simulink model "Adaptive_fuzzy_NTSMC"  (R2026a)
settings: Solver=FixedStepAuto  StopTime=150  FixedStep=0.005
values from neighbouring files (symbols this model uses):
  a1 = (Iy-Iz)/Ix    (= -0.733333333333)    [Initialization_3_Torque_Force.m]
  a2 = Jr/Ix    (= 0.008)    [Initialization_3_Torque_Force.m]
  a3 = (Iz-Ix)/Iy    (= 0.733333333333)    [Initialization_3_Torque_Force.m]
  a4 = Jr/Iy    (= 0.008)    [Initialization_3_Torque_Force.m]
  a5 = (Ix-Iy)/Iz    (= 0)    [Initialization_3_Torque_Force.m]
  beta_phi = beta    (= 2.5)    [Initialization_3_Torque_Force.m]
  beta_psi = beta    (= 2.5)    [Initialization_3_Torque_Force.m]
  beta_theta = beta    (= 2.5)    [Initialization_3_Torque_Force.m]
  distFactor = 19.0    (= 19)    [Initialization_3_Torque_Force.m]
  distMode = 3    [Initialization_3_Torque_Force.m]
  g = 9.8    [Initialization_3_Torque_Force.m]
  gama = 1.5    [Initialization_3_Torque_Force.m]
  Ix = 7.5e-3    (= 0.0075)    [Initialization_3_Torque_Force.m]
  Iy = 7.5e-3    (= 0.0075)    [Initialization_3_Torque_Force.m]
  Iz = 1.3e-2    (= 0.013)    [Initialization_3_Torque_Force.m]
  k_psi1 = 10    [Initialization_3_Torque_Force.m]
  k_psi2 = 10    [Initialization_3_Torque_Force.m]
  kd_x = -4    [Initialization_3_Torque_Force.m]
  kd_y = -4    [Initialization_3_Torque_Force.m]
  kd_z = -18    [Initialization_3_Torque_Force.m]
  kp_x = -3    [Initialization_3_Torque_Force.m]
  kp_y = -3    [Initialization_3_Torque_Force.m]
  kp_z = -12    [Initialization_3_Torque_Force.m]
  mass = 0.65    [Initialization_3_Torque_Force.m]
  ro = 0.3    [Initialization_3_Torque_Force.m]
  slctr = 3    [Initialization_3_Torque_Force.m]
  Tfinal = 150    [Initialization_3_Torque_Force.m]
  U2Omega = inv(Omega2U)    [Initialization_3_Torque_Force.m]
  w = [1 1 0.5]    [Initialization_3_Torque_Force.m]
  X0 = [10 10 5]    [Initialization_3_Torque_Force.m]
libraries: simulink x15, fuzblock x2, shared6dof x1
settings Model: Creator=elecomp  LastModifiedBy=asus

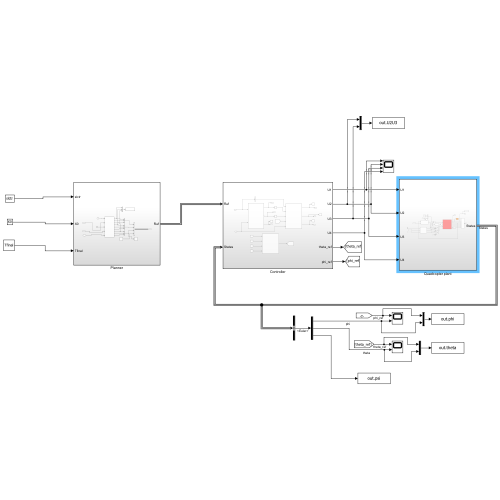
[thumbnail: Simulink's stored preview of the top-level diagram]
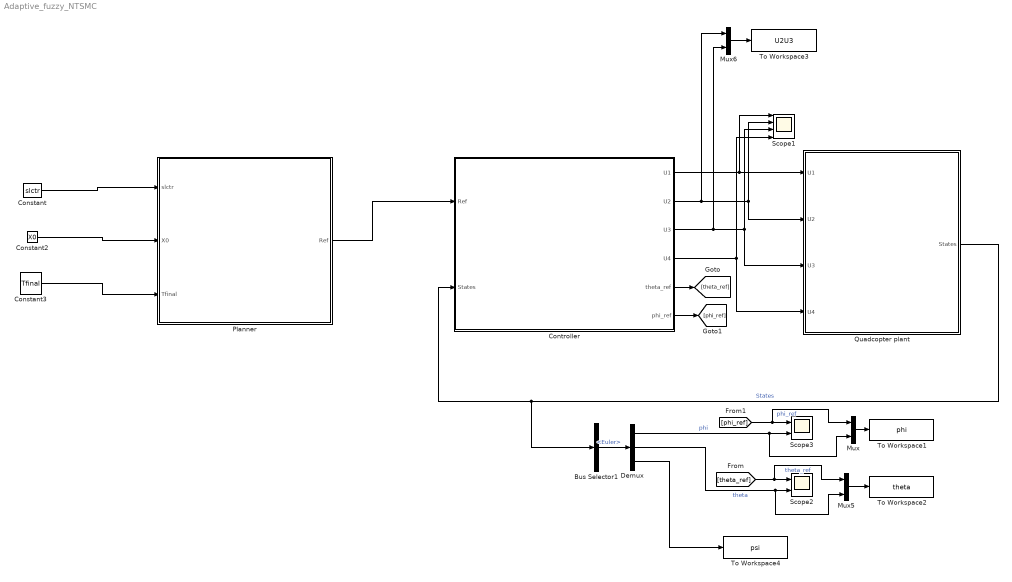
== system Adaptive_fuzzy_NTSMC ==
  Bus Selector1 : BusSelector  OutputSignals=Euler
  Constant : Constant  Value=slctr
  Constant2 : Constant  Value=X0
  Constant3 : Constant  Value=Tfinal
  Controller : Subsystem
  Demux : Demux  Outputs=3
  Mux : Mux  Inputs=2
  Mux5 : Mux  Inputs=2
  Mux6 : Mux  Inputs=2
  Planner : Subsystem
  Quadcopter plant : Subsystem
  Scope1 : Scope  NumInputPorts=4
      settings: ActiveDisplayYMinimum=-2.18019  ActiveDisplayYMaximum=1.22126  DataLoggingVariableName=ScopeData2
  Scope2 : Scope  NumInputPorts=2
      settings: ActiveDisplayYMinimum=-1.95741  ActiveDisplayYMaximum=1.91397
  Scope3 : Scope  NumInputPorts=2
      settings: ActiveDisplayYMinimum=-0.55732  ActiveDisplayYMaximum=1.11824  DataLoggingVariableName=ScopeData2
  To Workspace1 : ToWorkspace  VariableName=phi  SaveFormat=Timeseries  SampleTime=-1
  To Workspace2 : ToWorkspace  VariableName=theta  SaveFormat=Timeseries  SampleTime=-1
  To Workspace3 : ToWorkspace  VariableName=U2U3  SaveFormat=Timeseries  SampleTime=-1
  To Workspace4 : ToWorkspace  VariableName=psi  SaveFormat=Timeseries  SampleTime=-1
  wires:
  Quadcopter plant/1(States) -> Bus Selector1/1, Controller/2(States)  "States"
  Controller/1(U1) -> Scope1/1, Quadcopter plant/1(U1)
  Controller/2(U2) -> Mux6/1, Quadcopter plant/2(U2), Scope1/2
  Controller/3(U3) -> Mux6/2, Quadcopter plant/3(U3), Scope1/3
  Controller/4(U4) -> Quadcopter plant/4(U4), Scope1/4
  Bus Selector1/1 -> Demux/1  "<Euler>"
  Demux/2 -> Mux5/2, Scope2/2  "theta"
  Demux/1 -> Mux/2, Scope3/2  "phi"
  Controller/5(theta_ref) -> [theta_ref]
  Controller/6(phi_ref) -> [phi_ref]
  [theta_ref] -> Mux5/1, Scope2/1  "theta_ref"
  [phi_ref] -> Mux/1, Scope3/1  "phi_ref"
  Mux5/1 -> To Workspace2/1
  Mux/1 -> To Workspace1/1
  Mux6/1 -> To Workspace3/1
  Demux/3 -> To Workspace4/1
  Constant/1 -> Planner/1(slctr)
  Constant2/1 -> Planner/2(X0)
  Constant3/1 -> Planner/3(Tfinal)
  Planner/1(Ref) -> Controller/1(Ref)

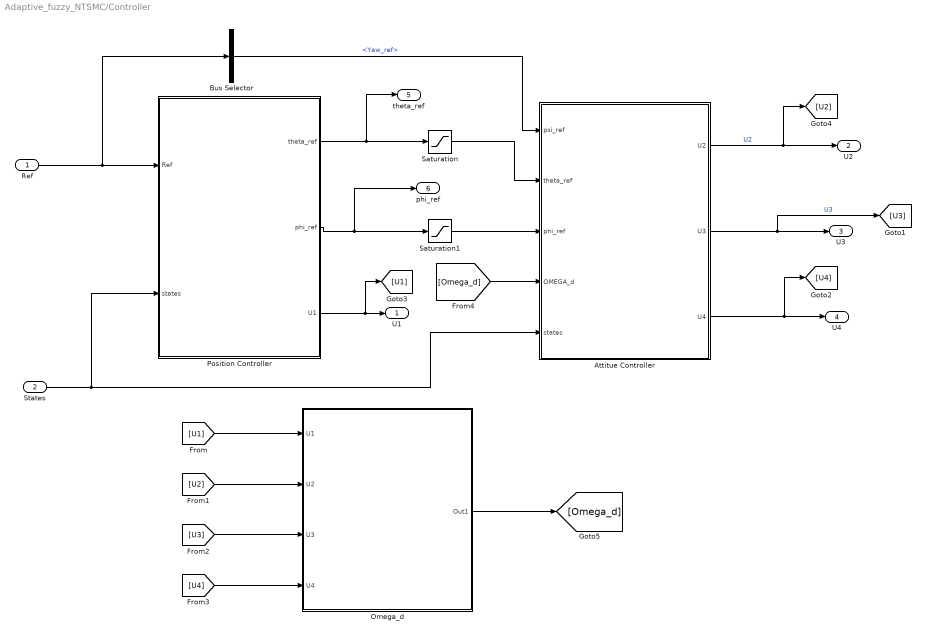
== system Adaptive_fuzzy_NTSMC/Controller ==
  Ref : Inport
  States : Inport  Port=2
  Attitue Controller : Subsystem
  Bus Selector : BusSelector  OutputSignals=Yaw_ref
  Omega_d : Subsystem
  Position Controller : Subsystem
  Saturation : Saturate  UpperLimit=0.7  LowerLimit=-0.7
  Saturation1 : Saturate  UpperLimit=0.7  LowerLimit=-0.7
  U1 : Outport
  U2 : Outport  Port=2
  U3 : Outport  Port=3
  U4 : Outport  Port=4
  theta_ref : Outport  Port=5
  phi_ref : Outport  Port=6
  wires:
  Ref/1 -> Bus Selector/1, Position Controller/1(Ref)
  Position Controller/3(U1) -> [U1], U1/1
  [Omega_d] -> Attitue Controller/4(OMEGA_d)
  Attitue Controller/1(U2) -> [U2], U2/1  "U2"
  Attitue Controller/2(U3) -> [U3], U3/1  "U3"
  Bus Selector/1 -> Attitue Controller/1(psi_ref)  "<Yaw_ref>"
  Attitue Controller/3(U4) -> [U4], U4/1
  Omega_d/1(Out1) -> [Omega_d]
  [U1] -> Omega_d/1(U1)
  [U2] -> Omega_d/2(U2)
  [U3] -> Omega_d/3(U3)
  [U4] -> Omega_d/4(U4)
  Position Controller/1(theta_ref) -> Saturation/1, theta_ref/1
  Position Controller/2(phi_ref) -> Saturation1/1, phi_ref/1
  States/1 -> Attitue Controller/5(states), Position Controller/2(states)
  Saturation/1 -> Attitue Controller/2(theta_ref)
  Saturation1/1 -> Attitue Controller/3(phi_ref)

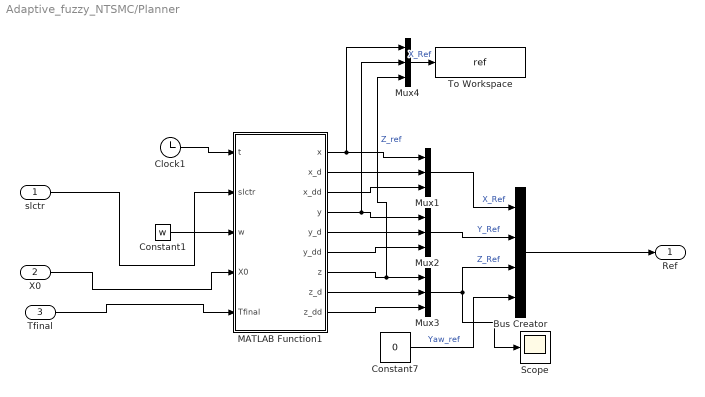
== system Adaptive_fuzzy_NTSMC/Planner ==
  slctr : Inport
  X0 : Inport  Port=2
  Tfinal : Inport  Port=3
  Bus Creator : BusCreator  Inputs=4
  Clock1 : Clock
  Constant1 : Constant  Value=w
  Constant7 : Constant  Value=0
  MATLAB Function1 : MATLAB Function  TreatAsAtomicUnit=on
  Mux{1..4} (4 alike) : Mux  Inputs=3
  Scope : Scope
      settings: ActiveDisplayYMinimum=-0.625  ActiveDisplayYMaximum=5.625
  To Workspace : ToWorkspace  VariableName=ref  SaveFormat=Timeseries  SampleTime=-1
  Ref : Outport
  wires:
  Constant7/1 -> Bus Creator/4  "Yaw_ref"
  MATLAB Function1/1(x) -> Mux4/1, Mux1/1
  MATLAB Function1/6(y_dd) -> Mux2/3
  MATLAB Function1/4(y) -> Mux4/2, Mux2/1
  Mux1/1 -> Bus Creator/1  "X_Ref"
  Mux3/1 -> Bus Creator/3, Scope/1  "Z_Ref"
  MATLAB Function1/3(x_dd) -> Mux1/3
  MATLAB Function1/7(z) -> Mux4/3, Mux3/1  "Z_ref"
  MATLAB Function1/9(z_dd) -> Mux3/3
  Bus Creator/1 -> Ref/1
  slctr/1 -> MATLAB Function1/2(slctr)
  Constant1/1 -> MATLAB Function1/3(w)
  Clock1/1 -> MATLAB Function1/1(t)
  MATLAB Function1/8(z_d) -> Mux3/2
  MATLAB Function1/2(x_d) -> Mux1/2
  Mux4/1 -> To Workspace/1  "X_Ref"
  MATLAB Function1/5(y_d) -> Mux2/2
  Mux2/1 -> Bus Creator/2  "Y_Ref"
  X0/1 -> MATLAB Function1/4(X0)
  Tfinal/1 -> MATLAB Function1/5(Tfinal)

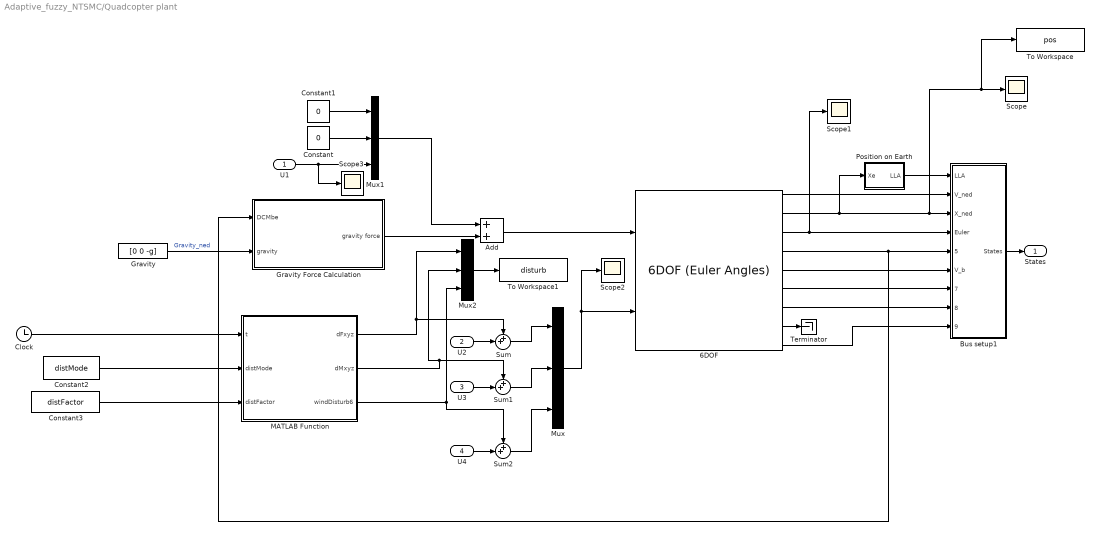
== system Adaptive_fuzzy_NTSMC/Quadcopter plant ==
  U1 : Inport
  U2 : Inport  Port=2
  U3 : Inport  Port=3
  U4 : Inport  Port=4
  "6DOF " : shared6dof/6DOF (Euler Angles)  units=Metric (MKS)  mtype=Fixed  rep=Euler Angles  xme_0=initpos  Vm_0=initvb  eul_0=initeuler  pm_0=initangRates  mass_0=mass  mass_e=0.5  mass_f=2.0  inertia=inertia_mat  inertia_e=eye(3)  inertia_f=2*eye(3)  k_quat=Vehicle.SixDOF.quatGain  vre_flag=on  abi_flag=on  aMode=aMode  xme_statename=''  Vm_statename=''  eul_statename=''  quat_statename=''  pm_statename=''  mass_statename=''
  Add : Sum
  Bus setup1 : Subsystem
  Clock : Clock
  Constant : Constant  Value=0
  Constant1 : Constant  Value=0
  Constant2 : Constant  Value=distMode
  Constant3 : Constant  Value=distFactor
  Gravity : Constant  Value=[0 0 -g]
  Gravity Force Calculation : Subsystem
  MATLAB Function : MATLAB Function  TreatAsAtomicUnit=on
  Mux : Mux  Inputs=3
  Mux1 : Mux  Inputs=3
  Mux2 : Mux  Inputs=3
  Position on Earth : Subsystem  Priority=1  TreatAsAtomicUnit=on
  Scope{,1..3} (4 alike) : Scope
      Scope settings: ActiveDisplayYMinimum=-12.55453  ActiveDisplayYMaximum=12.50157
      Scope1 settings: ActiveDisplayYMinimum=-0.86207  ActiveDisplayYMaximum=0.72361  DataLoggingVariableName=ScopeData4
      Scope2 settings: ActiveDisplayYMinimum=-0.018  ActiveDisplayYMaximum=0.05893  DataLoggingVariableName=ScopeData5
      Scope3 settings: ActiveDisplayYMinimum=-0.08846  ActiveDisplayYMaximum=0.08533
  Sum : Sum  Inputs=++|
  Sum1 : Sum  Inputs=++|
  Sum2 : Sum  Inputs=++|
  Terminator : Terminator
  To Workspace : ToWorkspace  VariableName=pos  SaveFormat=Timeseries  SampleTime=-1
  To Workspace1 : ToWorkspace  VariableName=disturb  SaveFormat=Timeseries  SampleTime=-1
  States : Outport
  wires:
  "6DOF "/4 -> Bus setup1/5(DCM_be), Gravity Force Calculation/1(DCMbe)
  Bus setup1/1(States) -> States/1
  "6DOF "/8 -> Terminator/1
  Gravity/1 -> Gravity Force Calculation/2(gravity)  "Gravity_ned"
  Mux/1 -> Scope2/1, "6DOF "/2
  U1/1 -> Scope3/1, Mux1/3
  Constant/1 -> Mux1/2
  Constant1/1 -> Mux1/1
  Gravity Force Calculation/1(gravity force) -> Add/2
  Mux1/1 -> Add/1
  Add/1 -> "6DOF "/1
  "6DOF "/1 -> Bus setup1/2(V_ned)
  "6DOF "/2 -> Position on Earth/1(Xe), To Workspace/1, Scope/1, Bus setup1/3(X_ned)
  "6DOF "/3 -> Bus setup1/4(Euler), Scope1/1
  "6DOF "/5 -> Bus setup1/6(V_b)
  "6DOF "/6 -> Bus setup1/7(Omega_b)
  "6DOF "/7 -> Bus setup1/8(dOmega_b)
  "6DOF "/9 -> Bus setup1/9(Accel_b)
  Position on Earth/1(LLA) -> Bus setup1/1(LLA)
  U4/1 -> Sum2/2
  U3/1 -> Sum1/2
  U2/1 -> Sum/2
  Sum/1 -> Mux/1
  Sum1/1 -> Mux/2
  Sum2/1 -> Mux/3
  MATLAB Function/3(windDisturb6) -> Sum2/1, Mux2/3
  Mux2/1 -> To Workspace1/1
  MATLAB Function/1(dFxyz) -> Mux2/1, Sum/1
  MATLAB Function/2(dMxyz) -> Mux2/2, Sum1/1
  Clock/1 -> MATLAB Function/1(t)
  Constant3/1 -> MATLAB Function/3(distFactor)
  Constant2/1 -> MATLAB Function/2(distMode)

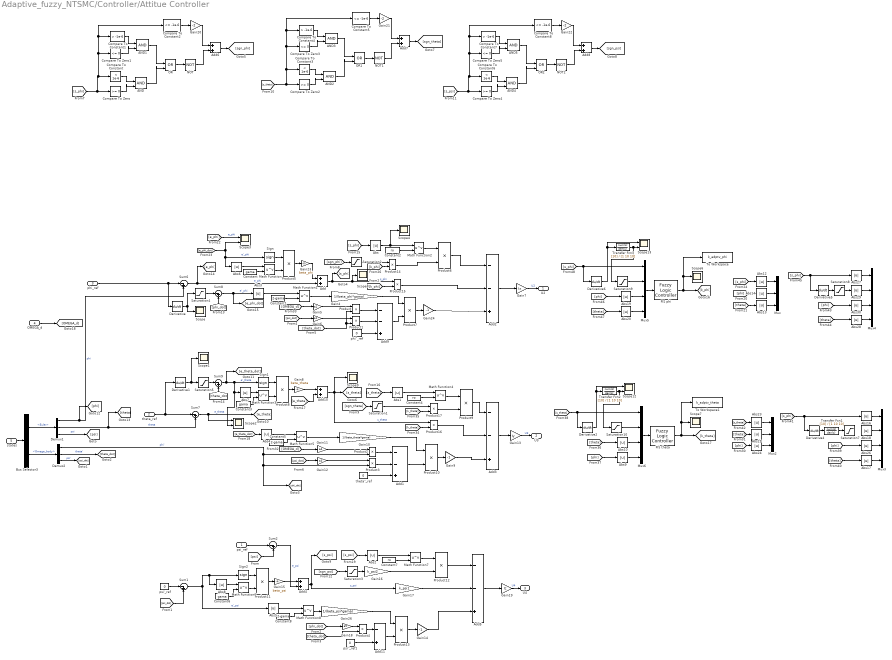
== system Adaptive_fuzzy_NTSMC/Controller/Attitue Controller ==
  psi_ref : Inport
  theta_ref : Inport  Port=2
  phi_ref : Inport  Port=3
  OMEGA_d : Inport  Port=4
  states : Inport  Port=5
  AND{,1..5} (6 alike) : Logic  IconShape=distinctive  AllPortsSameDT=off  OutDataTypeStr=boolean
  Abs{,1..10,12..14,16..20,23..30} (27 alike) : Abs  SaturateOnIntegerOverflow=off
  Add{,4,6..8,10} (6 alike) : Sum
  Add{1..3,5,9} (5 alike) : Sum  Inputs=--+
  Add11 : Sum  Inputs=-+
  Bus Selector3 : BusSelector  OutputSignals=Euler,Omega_body
  Compare To Constant : simulink/Logic and Bit Operations/Compare To Constant  relop=<  const=1e-6  OutDataTypeStr=boolean
  Compare To Constant1 : simulink/Logic and Bit Operations/Compare To Constant  relop=>  const=-1e-6  OutDataTypeStr=boolean
  Compare To Constant2 : simulink/Logic and Bit Operations/Compare To Constant  relop=<=  const=-1e-6  OutDataTypeStr=boolean
  Compare To Constant3 : simulink/Logic and Bit Operations/Compare To Constant  relop=<  const=1e-6  OutDataTypeStr=boolean
  Compare To Constant4 : simulink/Logic and Bit Operations/Compare To Constant  relop=>  const=-1e-6  OutDataTypeStr=boolean
  Compare To Constant5 : simulink/Logic and Bit Operations/Compare To Constant  relop=<=  const=-1e-6  OutDataTypeStr=boolean
  Compare To Constant6 : simulink/Logic and Bit Operations/Compare To Constant  relop=<  const=1e-6  OutDataTypeStr=boolean
  Compare To Constant7 : simulink/Logic and Bit Operations/Compare To Constant  relop=>  const=-1e-6  OutDataTypeStr=boolean
  Compare To Constant8 : simulink/Logic and Bit Operations/Compare To Constant  relop=<=  const=-1e-6  OutDataTypeStr=boolean
  Compare To Zero : simulink/Logic and Bit Operations/Compare To Zero  relop=>=  OutDataTypeStr=boolean
  Compare To Zero1 : simulink/Logic and Bit Operations/Compare To Zero  relop=<=  OutDataTypeStr=boolean
  Compare To Zero2 : simulink/Logic and Bit Operations/Compare To Zero  relop=>=  OutDataTypeStr=boolean
  Compare To Zero3 : simulink/Logic and Bit Operations/Compare To Zero  relop=<=  OutDataTypeStr=boolean
  Compare To Zero4 : simulink/Logic and Bit Operations/Compare To Zero  relop=>=  OutDataTypeStr=boolean
  Compare To Zero5 : simulink/Logic and Bit Operations/Compare To Zero  relop=<=  OutDataTypeStr=boolean
  Constant : Constant  Value=gama
  Constant1 : Constant  Value=2-gama
  Constant2 : Constant  Value=ro
  Constant3 : Constant  Value=gama
  Constant4 : Constant  Value=ro
  Constant5 : Constant  Value=2-gama
  Constant6 : Constant  Value=gama
  Constant7 : Constant  Value=ro
  Constant8 : Constant  Value=2-gama
  Demux1 : Demux  Outputs=3
  Demux2 : Demux  Outputs=3
  Derivative{,1..2,4..6} (6 alike) : Derivative
  FIS phi : fuzblock/Fuzzy Logic  Controller  FIS=fis_phi  OutputSampleNumber=101  DataType=double  UseLookupTable=off  NumBreakpoints=10  FuzzifiedInputs=off  RuleFiringStrengths=off  RuleOutputs=off  AggregatedOutputs=off  SimulateUsing=Interpreted execution  OutOfRangeInputValueMessage=warning  NoRuleFiredMessage=warning  EmptyOutputFuzzySetMessage=warning
  FIS theta : fuzblock/Fuzzy Logic  Controller  FIS=fis_theta  OutputSampleNumber=101  DataType=double  UseLookupTable=off  NumBreakpoints=10  FuzzifiedInputs=off  RuleFiringStrengths=off  RuleOutputs=off  AggregatedOutputs=off  SimulateUsing=Interpreted execution  OutOfRangeInputValueMessage=warning  NoRuleFiredMessage=warning  EmptyOutputFuzzySetMessage=warning
  Gain10 : Gain  Gain=1/(beta_theta*gama)
  Gain11 : Gain  Gain=a4
  Gain12 : Gain  Gain=a3
  Gain13 : Gain  Gain=Iy
  Gain14 : Gain  Gain=-1
  Gain15 : Gain  Gain=beta_psi
  Gain16 : Gain  Gain=k_psi2
  Gain17 : Gain  Gain=k_psi1
  Gain18 : Gain  Gain=a5
  Gain19 : Gain  Gain=Iz
  Gain20 : Gain  Gain=-2
  Gain21 : Gain  Gain=-2
  Gain22 : Gain  Gain=-2
  Gain23 : Gain  Gain=beta_phi
  Gain24 : Gain  Gain=-1
  Gain26 : Gain  Gain=1/(beta_psi*gama)
  Gain4 : Gain  Gain=1/(beta_phi*gama)
  Gain5 : Gain  Gain=a2
  Gain6 : Gain  Gain=a1
  Gain7 : Gain  Gain=Ix
  Gain8 : Gain  Gain=beta_theta
  Gain9 : Gain  Gain=-1
  Math Function{,1..8} (9 alike) : Math  Operator=pow
  Mux : Mux  Inputs=3
  Mux2 : Mux  Inputs=3
  Mux{3..6} (4 alike) : Mux
  NOT : Logic  Operator=NOT  IconShape=distinctive  AllPortsSameDT=off  OutDataTypeStr=boolean
  NOT1 : Logic  Operator=NOT  IconShape=distinctive  AllPortsSameDT=off  OutDataTypeStr=boolean
  NOT2 : Logic  Operator=NOT  IconShape=distinctive  AllPortsSameDT=off  OutDataTypeStr=boolean
  OR : Logic  Operator=OR  IconShape=distinctive  AllPortsSameDT=off  OutDataTypeStr=boolean
  OR1 : Logic  Operator=OR  IconShape=distinctive  AllPortsSameDT=off  OutDataTypeStr=boolean
  OR2 : Logic  Operator=OR  IconShape=distinctive  AllPortsSameDT=off  OutDataTypeStr=boolean
  Product{,1..17} (18 alike) : Product
  Saturation1 : Saturate  UpperLimit=1e-2  LowerLimit=-1e-2
  Saturation{4..5,7..10} (6 alike) : Saturate  UpperLimit=5  LowerLimit=-5
  Saturation2 : Saturate  UpperLimit=1e-2  LowerLimit=-1e-2
  Saturation3 : Saturate  UpperLimit=1e-2  LowerLimit=-1e-2
  Scope{,1,4,6..9} (7 alike) : Scope
      Scope settings: ActiveDisplayYMinimum=-3.5465  ActiveDisplayYMaximum=2.05103
      Scope1 settings: ActiveDisplayYMinimum=-1.87666  ActiveDisplayYMaximum=3.76434  DataLoggingVariableName=ScopeData3
      Scope4 settings: DataLoggingVariableName=ScopeData5
      Scope6 settings: ActiveDisplayYMinimum=10.04663  ActiveDisplayYMaximum=61.6606
      Scope7 settings: ActiveDisplayYMinimum=-2.98909  ActiveDisplayYMaximum=78.1099  DataLoggingVariableName=ScopeData2
      Scope8 settings: ActiveDisplayYMinimum=-0.44451  ActiveDisplayYMaximum=0.72337  DataLoggingVariableName=ScopeData3
      Scope9 settings: ActiveDisplayYMinimum=-0.27163  ActiveDisplayYMaximum=0.12798  DataLoggingVariableName=ScopeData4
  Scope{2..3,12..13} (4 alike) : Scope  NumInputPorts=2
      Scope12 settings: ActiveDisplayYMinimum=-1.41707  ActiveDisplayYMaximum=1.05628
      Scope13 settings: ActiveDisplayYMinimum=-0.35867  ActiveDisplayYMaximum=0.29003  DataLoggingVariableName=ScopeData2
      Scope2 settings: ActiveDisplayYMinimum=-1.13752  ActiveDisplayYMaximum=2.32672  DataLoggingVariableName=ScopeData3
      Scope3 settings: ActiveDisplayYMinimum=-0.92651  ActiveDisplayYMaximum=0.77112  DataLoggingVariableName=ScopeData4
  Sign : Signum
  Sign1 : Signum
  Sign2 : Signum
  Sum{1..2,6..9} (6 alike) : Sum  Inputs=|-+
  To Workspace : ToWorkspace  VariableName=k_adptv_phi  SaveFormat=Timeseries  SampleTime=-1
  To Workspace1 : ToWorkspace  VariableName=k_adptv_theta  SaveFormat=Timeseries  SampleTime=-1
  Transfer Fcn1 : TransferFcn  Numerator=[10]  Denominator=[1 10 10]
  Transfer Fcn2 : TransferFcn  Numerator=[10]  Denominator=[1 10 10]
  Transfer Fcn3 : TransferFcn  Numerator=[10]  Denominator=[1 10 10]
  phi''_ref : Constant  Value=0
  psi''_ref1 : Constant  Value=0
  psi'_ref : Constant  Value=0
  theta''_ref : Constant  Value=0
  U2 : Outport
  U3 : Outport  Port=2
  U4 : Outport  Port=3
  wires:
  Sum6/1 -> Add/2, [e_phi]  "e_phi"
  Demux1/2 -> [theta], Sum7/2  "theta"
  Saturation2/1 -> Product14/1
  Gain12/1 -> Product3/1
  Add2/1 -> Gain7/1
  Product15/1 -> Add2/2
  Gain13/1 -> U3/1  "U3"
  Add3/1 -> Gain13/1
  Sum7/1 -> Scope2/1, [e_theta]  "e_theta"
  Sum8/1 -> [e_phi_dot], Abs3/1  "e'_phi"
  Demux2/3 -> [psi_dot]  "psi'"
  Gain5/1 -> Product/1
  Add/1 -> Scope8/1, Product15/1, [s_phi]  "s_phi"
  Gain6/1 -> Product1/1
  Gain7/1 -> U2/1  "U2"
  Demux1/1 -> [phi], Sum6/2  "phi"
  Bus Selector3/1 -> Demux1/1  "<Euler>"
  Gain11/1 -> Product2/1
  states/1 -> Bus Selector3/1
  Demux1/3 -> [psi]  "psi"
  Bus Selector3/2 -> Demux2/1  "<Omega_body>"
  Demux2/1 -> Product3/2, [phi_dot], Product2/2  "phi'"
  Demux2/2 -> [theta_dot]  "theta'"
  psi'_ref/1 -> Sum1/1
  psi_ref/1 -> Sum2/1
  [psi] -> Sum2/2
  Sum2/1 -> Add4/2  "e_psi"
  [psi_dot] -> Sum1/2
  Gain18/1 -> Product4/1
  [theta_dot] -> Product4/2
  [phi_dot] -> Gain18/1
  Gain19/1 -> U4/1  "U4"
  Add5/1 -> Gain19/1
  [psi_dot] -> Gain6/1
  [theta_dot] -> Product/2, Product1/2
  [psi_dot] -> Gain12/1
  phi_ref/1 -> Sum6/1, Derivative/1
  theta_ref/1 -> Sum7/1, Derivative1/1
  Compare To Zero/1 -> AND/2
  Compare To Constant/1 -> AND/1
  Compare To Constant1/1 -> AND1/1
  Compare To Zero1/1 -> AND1/2
  AND1/1 -> OR/1
  AND/1 -> OR/2
  OR/1 -> NOT/1
  Compare To Constant2/1 -> Gain20/1
  NOT/1 -> Add6/2
  Gain20/1 -> Add6/1
  [s_phi] -> Compare To Constant2/1, Compare To Constant1/1, Compare To Zero1/1, Compare To Constant/1, Compare To Zero/1
  Add6/1 -> [sgn_phi]
  [sgn_phi] -> Saturation2/1
  Add7/1 -> [sgn_theta]
  [s_theta] -> Compare To Zero2/1, Compare To Constant3/1, Compare To Zero3/1, Compare To Constant4/1, Compare To Constant5/1
  Gain21/1 -> Add7/1
  NOT1/1 -> Add7/2
  Compare To Constant5/1 -> Gain21/1
  OR1/1 -> NOT1/1
  AND2/1 -> OR1/2
  AND3/1 -> OR1/1
  Compare To Zero3/1 -> AND3/2
  Compare To Constant4/1 -> AND3/1
  Compare To Constant3/1 -> AND2/1
  Compare To Zero2/1 -> AND2/2
  Compare To Zero4/1 -> AND4/2
  Compare To Constant6/1 -> AND4/1
  Compare To Constant7/1 -> AND5/1
  Compare To Zero5/1 -> AND5/2
  AND5/1 -> OR2/1
  AND4/1 -> OR2/2
  OR2/1 -> NOT2/1
  Compare To Constant8/1 -> Gain22/1
  NOT2/1 -> Add8/2
  Gain22/1 -> Add8/1
  [s_psi] -> Compare To Constant8/1, Compare To Constant7/1, Compare To Zero5/1, Compare To Constant6/1, Compare To Zero4/1
  Add8/1 -> [sgn_psi]
  Constant/1 -> Math Function/2
  Math Function/1 -> Product5/2
  Product5/1 -> Gain23/1
  Sign/1 -> Product5/1
  [phi_dot] -> Sum8/2
  [theta_dot] -> Sum9/2
  Gain23/1 -> Add/1
  Product6/1 -> Add2/1
  [s_phi] -> Abs/1
  Product/1 -> Add9/1
  Product1/1 -> Add9/2
  phi''_ref/1 -> Add9/3
  Gain4/1 -> Product7/1
  Add9/1 -> Product7/2
  Product7/1 -> Gain24/1
  Gain24/1 -> Add2/3
  Math Function1/1 -> Gain4/1
  Constant1/1 -> Math Function1/2
  Abs/1 -> Scope4/1, Math Function2/1
  Constant2/1 -> Math Function2/2
  Math Function2/1 -> Product6/1
  Product2/1 -> Add1/1
  Product3/1 -> Add1/2
  theta''_ref/1 -> Add1/3
  Sign1/1 -> Product8/1
  Product8/1 -> Gain8/1
  Math Function3/1 -> Product8/2
  Constant3/1 -> Math Function3/2
  Sum9/1 -> [e_theta_dot], Scope2/2, Abs7/1, Sign1/1  "e'_theta"
  Gain8/1 -> Add10/1
  Add10/1 -> Scope9/1, Product16/1, [s_theta]  "s_theta"
  Math Function4/1 -> Product9/1
  Constant4/1 -> Math Function4/2
  Abs1/1 -> Math Function4/1
  [s_theta] -> Abs1/1
  [sgn_theta] -> Saturation1/1
  [e_theta] -> Add10/2
  Product10/1 -> Gain9/1
  Add1/1 -> Product10/2
  Constant5/1 -> Math Function5/2
  Math Function5/1 -> Gain10/1
  Gain10/1 -> Product10/1
  Product9/1 -> Add3/1
  Product16/1 -> Add3/2
  Gain9/1 -> Add3/3
  Product4/1 -> Add11/1
  psi''_ref1/1 -> Add11/2
  Gain15/1 -> Add4/1
  Constant6/1 -> Math Function6/2
  Math Function6/1 -> Product11/2
  Product11/1 -> Gain15/1
  Sum1/1 -> Abs5/1, Sign2/1, Abs8/1  "e'_psi"
  Sign2/1 -> Product11/1
  Add4/1 -> [s_psi], Gain17/1  "s_psi"
  Saturation3/1 -> Gain16/1
  [sgn_psi] -> Saturation3/1
  Gain16/1 -> Product12/2
  [s_psi] -> Abs2/1
  Abs2/1 -> Math Function7/1
  Constant7/1 -> Math Function7/2
  Math Function7/1 -> Product12/1
  Product12/1 -> Add5/1
  Gain17/1 -> Add5/2
  Gain14/1 -> Add5/3
  Abs3/1 -> Math Function1/1
  [e_theta_dot] -> Abs4/1
  Abs4/1 -> Math Function5/1
  Add11/1 -> Product13/2
  Product13/1 -> Gain14/1
  Gain26/1 -> Product13/1
  Abs5/1 -> Math Function8/1
  Constant8/1 -> Math Function8/2
  Math Function8/1 -> Gain26/1
  Abs6/1 -> Math Function/1
  Abs7/1 -> Math Function3/1
  Abs8/1 -> Math Function6/1
  Saturation4/1 -> Sum8/1
  Derivative1/1 -> Saturation5/1, Scope1/1
  Saturation5/1 -> Sum9/1
  Derivative/1 -> Saturation4/1, Scope/1
  [e_phi] -> Scope3/1  "e_phi"
  [e_phi_dot] -> Abs6/1, Sign/1, Scope3/2  "e'_phi"
  FIS phi/1 -> To Workspace/1, Scope6/1, [k_phi]
  Product14/1 -> Product6/2
  [k_phi] -> Product14/2
  [k_phi] -> Product15/2
  FIS theta/1 -> [k_theta], To Workspace1/1, Scope7/1
  OMEGA_d/1 -> [OMEGA_d]
  [OMEGA_d] -> Gain11/1
  [OMEGA_d] -> Gain5/1
  [k_theta] -> Product16/2
  Saturation1/1 -> Product17/1
  Product17/1 -> Product9/2
  [k_theta] -> Product17/2
  [theta] -> Abs13/1
  [s_phi] -> Abs12/1
  [phi] -> Abs14/1
  [phi] -> Abs24/1
  [theta] -> Abs25/1
  [s_theta] -> Abs23/1
  [s_phi] -> Derivative4/1, Abs16/1
  [phi] -> Abs26/1
  [theta] -> Abs17/1
  Abs16/1 -> Mux3/1
  Abs18/1 -> Mux3/2
  Abs26/1 -> Mux3/3
  Abs17/1 -> Mux3/4
  Transfer Fcn1/1 -> Saturation7/1
  Derivative4/1 -> Transfer Fcn1/1
  Saturation8/1 -> Abs29/1
  Derivative5/1 -> Saturation8/1
  Abs29/1 -> Mux4/2
  Abs28/1 -> Mux4/4
  Abs30/1 -> Mux4/3
  [theta] -> Abs28/1
  Abs27/1 -> Mux4/1
  [s_phi] -> Derivative5/1, Abs27/1
  [phi] -> Abs30/1
  Abs19/1 -> Mux5/3
  Abs20/1 -> Mux5/4
  Transfer Fcn3/1 -> Scope13/2, Saturation9/1
  Derivative6/1 -> Transfer Fcn3/1, Scope13/1
  Saturation9/1 -> Mux5/2
  [theta] -> Abs20/1
  [phi] -> Abs19/1
  [s_phi] -> Derivative6/1, Mux5/1
  Abs13/1 -> Mux/3
  Abs14/1 -> Mux/2
  Abs12/1 -> Mux/1
  Abs24/1 -> Mux2/3
  Abs25/1 -> Mux2/2
  Abs23/1 -> Mux2/1
  Abs10/1 -> Mux6/3
  Abs9/1 -> Mux6/4
  Transfer Fcn2/1 -> Scope12/2, Saturation10/1
  Derivative2/1 -> Transfer Fcn2/1, Scope12/1
  [phi] -> Abs9/1
  [s_theta] -> Derivative2/1, Mux6/1
  Saturation10/1 -> Mux6/2
  [theta] -> Abs10/1
  Mux5/1 -> FIS phi/1
  Mux6/1 -> FIS theta/1

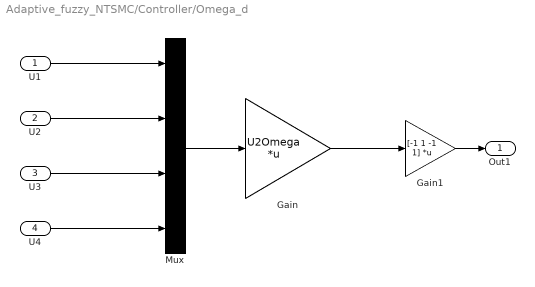
== system Adaptive_fuzzy_NTSMC/Controller/Omega_d ==
  U1 : Inport
  U2 : Inport  Port=2
  U3 : Inport  Port=3
  U4 : Inport  Port=4
  Gain : Gain  Gain=U2Omega  Multiplication=Matrix(K*u)
  Gain1 : Gain  Gain=[-1 1 -1 1]  Multiplication=Matrix(K*u)
  Mux : Mux
  Out1 : Outport
  wires:
  U3/1 -> Mux/3
  Mux/1 -> Gain/1
  U4/1 -> Mux/4
  U1/1 -> Mux/1
  U2/1 -> Mux/2
  Gain/1 -> Gain1/1
  Gain1/1 -> Out1/1

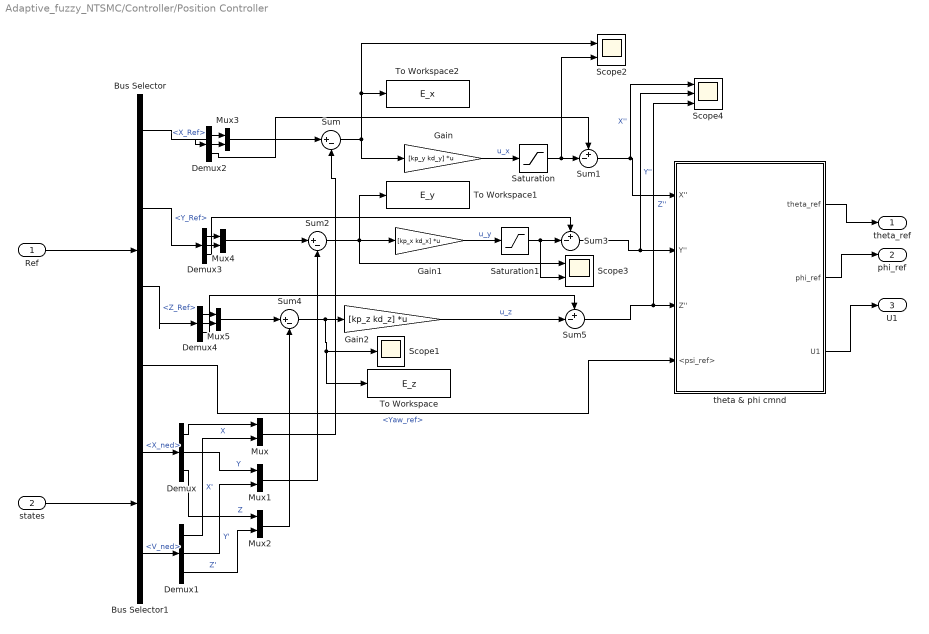
== system Adaptive_fuzzy_NTSMC/Controller/Position Controller ==
  Ref : Inport
  states : Inport  Port=2
  Bus Selector : BusSelector  OutputSignals=X_Ref,Y_Ref,Z_Ref,Yaw_ref
  Bus Selector1 : BusSelector  OutputSignals=X_ned,V_ned
  Demux{,1..4} (5 alike) : Demux  Outputs=3
  Gain : Gain  Gain=[kp_y kd_y]  Multiplication=Matrix(K*u)
  Gain1 : Gain  Gain=[kp_x kd_x]  Multiplication=Matrix(K*u)
  Gain2 : Gain  Gain=[kp_z kd_z]  Multiplication=Matrix(K*u)
  Mux{,1..5} (6 alike) : Mux  Inputs=2
  Saturation : Saturate  UpperLimit=8  LowerLimit=-8
  Saturation1 : Saturate  UpperLimit=8  LowerLimit=-8
  Scope1 : Scope
      settings: ActiveDisplayYMinimum=-10.24452  ActiveDisplayYMaximum=10.02717
  Scope2 : Scope  NumInputPorts=2
      settings: ActiveDisplayYMinimum=-6.33993  ActiveDisplayYMaximum=3.48221  DataLoggingVariableName=ScopeData2
  Scope3 : Scope  NumInputPorts=2
      settings: ActiveDisplayYMinimum=-9.625  ActiveDisplayYMaximum=6.625  DataLoggingVariableName=ScopeData3
  Scope4 : Scope  NumInputPorts=3
      settings: ActiveDisplayYMinimum=-28.74037  ActiveDisplayYMaximum=28.88937  DataLoggingVariableName=ScopeData2
  Sum : Sum  Inputs=|+-
  Sum1 : Sum  Inputs=+-|
  Sum2 : Sum  Inputs=|+-
  Sum3 : Sum  Inputs=+-|
  Sum4 : Sum  Inputs=|+-
  Sum5 : Sum  Inputs=+-|
  To Workspace : ToWorkspace  VariableName=E_z  SaveFormat=Timeseries  SampleTime=-1
  To Workspace1 : ToWorkspace  VariableName=E_y  SaveFormat=Timeseries  SampleTime=-1
  To Workspace2 : ToWorkspace  VariableName=E_x  SaveFormat=Timeseries  SampleTime=-1
  theta & phi cmnd : Subsystem
  theta_ref : Outport
  phi_ref : Outport  Port=2
  U1 : Outport  Port=3
  wires:
  Sum5/1 -> Scope4/3, theta & phi cmnd/3(Z'')  "Z''"
  Bus Selector/3 -> Demux4/1  "<Z_Ref>"
  Bus Selector1/1 -> Demux/1  "<X_ned>"
  Bus Selector/2 -> Demux3/1  "<Y_Ref>"
  Ref/1 -> Bus Selector/1
  Sum1/1 -> Scope4/1, theta & phi cmnd/1(X'')  "X''"
  theta & phi cmnd/2(phi_ref) -> phi_ref/1
  Gain1/1 -> Saturation1/1  "u_y"
  Gain2/1 -> Sum5/2  "u_z"
  Sum3/1 -> Scope4/2, theta & phi cmnd/2(Y'')  "Y''"
  Gain/1 -> Saturation/1  "u_x"
  theta & phi cmnd/1(theta_ref) -> theta_ref/1
  Bus Selector/1 -> Demux2/1  "<X_Ref>"
  Bus Selector/4 -> theta & phi cmnd/4(<psi_ref>)  "<Yaw_ref>"
  theta & phi cmnd/3(U1) -> U1/1
  states/1 -> Bus Selector1/1
  Demux/1 -> Mux/1  "X"
  Bus Selector1/2 -> Demux1/1  "<V_ned>"
  Demux1/1 -> Mux/2  "X'"
  Demux/2 -> Mux1/1  "Y"
  Demux1/2 -> Mux1/2  "Y'"
  Demux1/3 -> Mux2/2  "Z'"
  Demux/3 -> Mux2/1  "Z"
  Mux/1 -> Sum/2
  Mux1/1 -> Sum2/2
  Mux2/1 -> Sum4/2
  Demux2/3 -> Sum1/1
  Demux3/3 -> Sum3/1
  Demux4/3 -> Sum5/1
  Demux2/1 -> Mux3/1
  Demux2/2 -> Mux3/2
  Mux3/1 -> Sum/1
  Demux3/1 -> Mux4/1
  Demux3/2 -> Mux4/2
  Mux4/1 -> Sum2/1
  Demux4/1 -> Mux5/1
  Demux4/2 -> Mux5/2
  Mux5/1 -> Sum4/1
  Sum/1 -> Gain/1, To Workspace2/1, Scope2/1
  Sum2/1 -> To Workspace1/1, Scope3/1, Gain1/1
  Sum4/1 -> To Workspace/1, Scope1/1, Gain2/1
  Saturation/1 -> Scope2/2, Sum1/2
  Saturation1/1 -> Scope3/2, Sum3/2

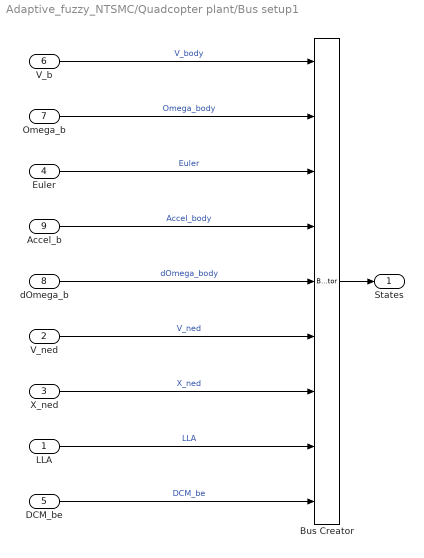
== system Adaptive_fuzzy_NTSMC/Quadcopter plant/Bus setup1 ==
  LLA : Inport  PortDimensions=3
  V_ned : Inport  Port=2  Unit=m/second  PortDimensions=3
  X_ned : Inport  Port=3  Unit=m  PortDimensions=3
  Euler : Inport  Port=4  Unit=rad  PortDimensions=3
  DCM_be : Inport  Port=5  PortDimensions=[3 3]
  V_b : Inport  Port=6  Unit=m/s  PortDimensions=3
  Omega_b : Inport  Port=7  Unit=rad/s  PortDimensions=3
  dOmega_b : Inport  Port=8  Unit=rad/s^2  PortDimensions=3
  Accel_b : Inport  Port=9  Unit=m/s^2  PortDimensions=3
  Bus Creator : BusCreator  Inputs=9
  States : Outport  VectorParamsAs1DForOutWhenUnconnected=off
  wires:
  V_b/1 -> Bus Creator/1  "V_body"
  Omega_b/1 -> Bus Creator/2  "Omega_body"
  Euler/1 -> Bus Creator/3  "Euler"
  X_ned/1 -> Bus Creator/7  "X_ned"
  Accel_b/1 -> Bus Creator/4  "Accel_body"
  LLA/1 -> Bus Creator/8  "LLA"
  dOmega_b/1 -> Bus Creator/5  "dOmega_body"
  DCM_be/1 -> Bus Creator/9  "DCM_be"
  V_ned/1 -> Bus Creator/6  "V_ned"
  Bus Creator/1 -> States/1

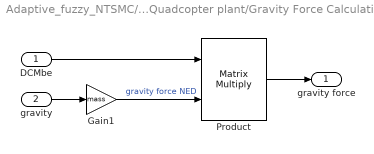
== system Adaptive_fuzzy_NTSMC/Quadcopter plant/Gravity Force Calculation ==
  DCMbe : Inport
  gravity : Inport  Port=2  Unit=m/s^2
  Gain1 : Gain  Gain=mass
  Product : Product  Multiplication=Matrix(*)
  gravity force : Outport  Unit=N  VectorParamsAs1DForOutWhenUnconnected=off
  wires:
  gravity/1 -> Gain1/1
  Gain1/1 -> Product/2  "gravity force NED"
  Product/1 -> gravity force/1
  DCMbe/1 -> Product/1

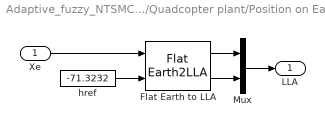
== system Adaptive_fuzzy_NTSMC/Quadcopter plant/Position on Earth ==
  Xe : Inport  Unit=m
  Flat Earth to LLA : FlatEarth2LLA  R=6378137  LL0="[42.2999  -71.3504]"
  Mux : Mux  Inputs=2
  href : Constant  Value=-71.3232
  LLA : Outport  VectorParamsAs1DForOutWhenUnconnected=off
  wires:
  Mux/1 -> LLA/1
  Xe/1 -> Flat Earth to LLA/1
  Flat Earth to LLA/1 -> Mux/1
  Flat Earth to LLA/2 -> Mux/2
  href/1 -> Flat Earth to LLA/2

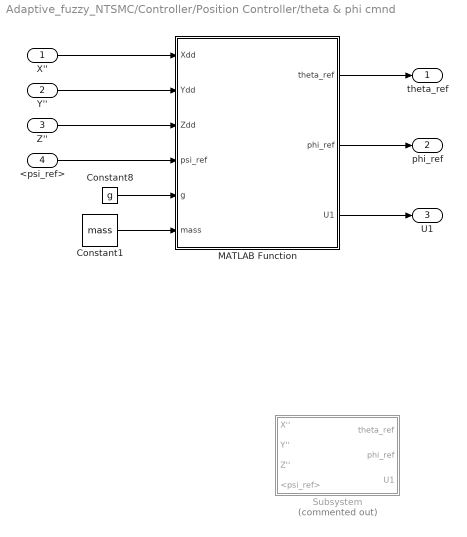
== system Adaptive_fuzzy_NTSMC/Controller/Position Controller/theta & phi cmnd ==
  X'' : Inport
  Y'' : Inport  Port=2
  Z'' : Inport  Port=3
  <psi_ref> : Inport  Port=4
  Constant1 : Constant  Value=mass
  Constant8 : Constant  Value=g
  MATLAB Function : MATLAB Function  TreatAsAtomicUnit=on
  Subsystem : Subsystem  Commented=on
  theta_ref : Outport
  phi_ref : Outport  Port=2
  U1 : Outport  Port=3
  wires:
  X''/1 -> MATLAB Function/1(Xdd)
  Y''/1 -> MATLAB Function/2(Ydd)
  Z''/1 -> MATLAB Function/3(Zdd)
  <psi_ref>/1 -> MATLAB Function/4(psi_ref)
  Constant8/1 -> MATLAB Function/5(g)
  Constant1/1 -> MATLAB Function/6(mass)
  MATLAB Function/1(theta_ref) -> theta_ref/1
  MATLAB Function/2(phi_ref) -> phi_ref/1
  MATLAB Function/3(U1) -> U1/1

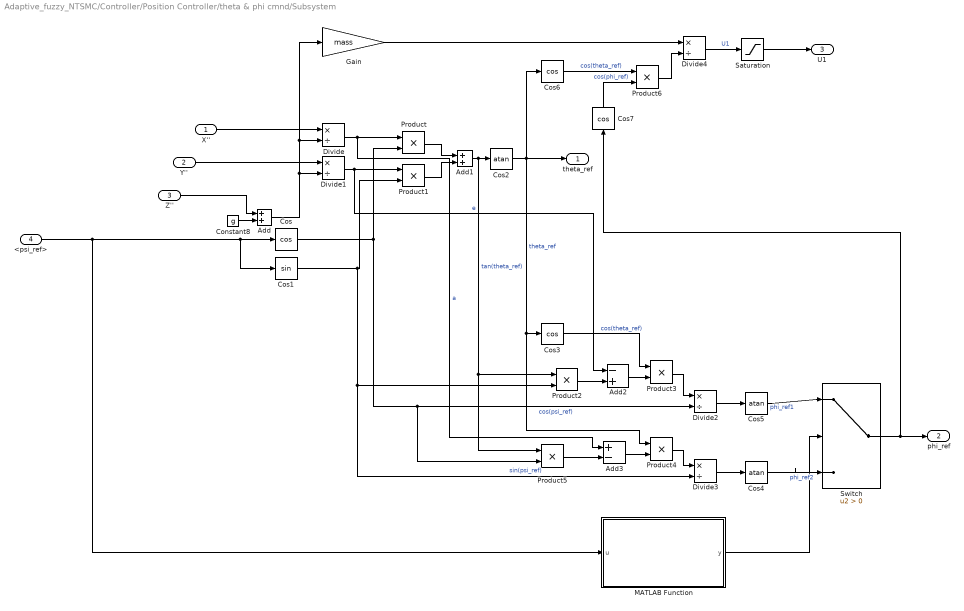
== system Adaptive_fuzzy_NTSMC/Controller/Position Controller/theta & phi cmnd/Subsystem ==
  X'' : Inport
  Y'' : Inport  Port=2
  Z'' : Inport  Port=3
  <psi_ref> : Inport  Port=4
  Add : Sum
  Add1 : Sum
  Add2 : Sum  Inputs=-+
  Add3 : Sum  Inputs=+-
  Constant8 : Constant  Value=g
  Cos : Trigonometry  Operator=cos
  Cos1 : Trigonometry
  Cos2 : Trigonometry  Operator=atan  OutputSignalType=real
  Cos3 : Trigonometry  Operator=cos  OutputSignalType=real
  Cos4 : Trigonometry  Operator=atan  OutputSignalType=real
  Cos5 : Trigonometry  Operator=atan  OutputSignalType=real
  Cos6 : Trigonometry  Operator=cos  OutputSignalType=real
  Cos7 : Trigonometry  Operator=cos  OutputSignalType=real
  Divide{,1..4} (5 alike) : Product  Inputs=*/
  Gain : Gain  Gain=mass
  MATLAB Function : MATLAB Function  TreatAsAtomicUnit=on
  Product{,1..6} (7 alike) : Product
  Saturation : Saturate  UpperLimit=inf  LowerLimit=0
  Switch : Switch  Criteria=u2 > Threshold  SaturateOnIntegerOverflow=off  InputSameDT=off
  theta_ref : Outport
  phi_ref : Outport  Port=2
  U1 : Outport  Port=3
  wires:
  Saturation/1 -> U1/1
  <psi_ref>/1 -> MATLAB Function/1(u), Cos1/1, Cos/1
  Add1/1 -> Product5/1, Product2/1, Cos2/1  "tan(theta_ref)"
  Cos/1 -> Product/2, Product5/2, Divide2/2  "cos(psi_ref)"
  Product1/1 -> Add1/2
  Switch/1 -> phi_ref/1, Cos7/1
  Add/1 -> Divide1/2, Gain/1, Divide/2
  Product2/1 -> Add2/2
  Cos4/1 -> Switch/3  "phi_ref2"
  X''/1 -> Divide/1
  Cos1/1 -> Divide3/2, Product2/2, Product1/2  "sin(psi_ref)"
  Constant8/1 -> Add/2
  Cos2/1 -> theta_ref/1, Cos6/1, Product4/1, Cos3/1  "theta_ref"
  Y''/1 -> Divide1/1
  Z''/1 -> Add/1
  Divide1/1 -> Add2/1, Product1/1  "e"
  Add3/1 -> Product4/2
  Divide2/1 -> Cos5/1
  Divide/1 -> Add3/1, Product/1  "a"
  Cos3/1 -> Product3/1  "cos(theta_ref)"
  Product3/1 -> Divide2/1
  Cos7/1 -> Product6/2  "cos(phi_ref)"
  Product4/1 -> Divide3/1
  Cos5/1 -> Switch/1  "phi_ref1"
  MATLAB Function/1(y) -> Switch/2
  Divide4/1 -> Saturation/1  "U1"
  Product6/1 -> Divide4/2
  Divide3/1 -> Cos4/1
  Product5/1 -> Add3/2
  Add2/1 -> Product3/2
  Product/1 -> Add1/1
  Cos6/1 -> Product6/1  "cos(theta_ref)"
  Gain/1 -> Divide4/1

== matlab function Adaptive_fuzzy_NTSMC/Controller/Position Controller/theta & phi cmnd/MATLAB Function ==
  data: Xdd input; theta_ref output; Ydd input; Zdd input; psi_ref input; g input; mass input; phi_ref output; U1 output
function [theta_ref, phi_ref, U1] = fcn(Xdd, Ydd, Zdd, psi_ref , g, mass)

theta_ref = atan( (Xdd / (Zdd+g))*cos(psi_ref) + (Ydd / (Zdd+g))*sin(psi_ref) );

if psi_ref>=0 & psi_ref<pi/4
    phi_ref = atan( cos(theta_ref) * ( tan(theta_ref)*sin(psi_ref) - (Ydd / (Zdd+g))) / (cos(psi_ref)) );
elseif psi_ref<=2*pi & psi_ref<7*pi/4
    phi_ref = atan( cos(theta_ref) * ( tan(theta_ref)*sin(psi_ref) - (Ydd / (Zdd+g))) / (cos(psi_ref)) );
elseif psi_ref>=3*pi/4 & psi_ref<5*pi/4
    phi_ref = atan( cos(theta_ref) * ( tan(theta_ref)*sin(psi_ref) - (Ydd / (Zdd+g))) / (cos(psi_ref)) );

elseif psi_ref>pi/4 & psi_ref<3*pi/4
    phi_ref = atan( cos(theta_ref) * ( (Xdd / (Zdd+g)) - tan(theta_ref)*cos(psi_ref) ) / (sin(psi_ref)) );
else
    phi_ref = atan( cos(theta_ref) * ( (Xdd / (Zdd+g)) - tan(theta_ref)*cos(psi_ref) ) / (sin(psi_ref)) );
end

% phi_ref = -abs(phi_ref);

U1 = mass * (Zdd+g) / (cos(phi_ref)*cos(psi_ref));

end

== matlab function Adaptive_fuzzy_NTSMC/Controller/Position Controller/theta & phi cmnd/Subsystem/MATLAB Function ==
  data: u input; y output
function y = fcn(u)

if u>=0 & u<pi/4
    y=1;
elseif u<=2*pi & u<7*pi/4
    y=1;
elseif u>=3*pi/4 & u<5*pi/4
    y=1;
elseif u>pi/4 & u<3*pi/4
    y=0;
else
    y=0;
end
end

== matlab function Adaptive_fuzzy_NTSMC/Quadcopter plant/MATLAB Function ==
  data: t input; dFxyz output; distMode input; distFactor input; dMxyz output; windDisturb6 output
function [dFxyz, dMxyz, windDisturb6] = fcn(t, distMode, distFactor)
% Paper-style wind/gust disturbance generator for the CURRENT model wiring.
%
% IMPORTANT FOR YOUR CURRENT SIMULINK MODEL:
% This version uses SCALAR outputs, so you do NOT need Demux blocks and you
% do NOT need to change the plant force input wiring.
%
% Output-port usage for your current wiring:
%   dFxyz        -> connect to the U2 add block  = roll moment disturbance
%   dMxyz        -> connect to the U3 add block  = pitch moment disturbance
%   windDisturb6 -> connect to the U4 add block  = yaw moment disturbance
%
% Inputs:
%   t          : Clock signal, seconds
%   distMode   : 0=off, 1=mild, 2=paper/strong, 3=custom
%   distFactor : multiplier for all disturbance amplitudes
%
% Paper-style disturbance shape:
%   - step/gust impacts at 6 s, 10 s, and 15 s
%   - sinusoidal airflow at 0.5 Hz from 20 s to 30 s
%
% Note:
% The paper describes angular disturbances. In this 6DOF plant, the same
% time profile is converted to small moment disturbances in N.m.

mode = round(distMode);
if mode < 0
    mode = 0;
end

factor = abs(distFactor);

% ------------------------------------------------------------
% Paper-style timing and normalized amplitudes
% ------------------------------------------------------------
stepAmpPaper = 1.5;       % normalized step/gust amplitude from paper
sineAmpPaper = 1.0;       % normalized sine amplitude from paper
sineFreqHz   = 0.5;       % paper sine frequency, Hz
sineOmega    = 2*pi*sineFreqHz;

t1 = 6.0;
t2 = 10.0;
t3 = 15.0;
gustWidth = 0.80;         % seconds, gust pulse duration

sineStart = 20.0;
sineEnd   = 30.0;

% ------------------------------------------------------------
% Convert normalized paper disturbance to moment disturbance.
% Use distMode = 2 for the closest paper-like strong test.
% ------------------------------------------------------------
if mode == 0
    M_step_scale = 0.0;
    M_sine_scale = 0.0;
elseif mode == 1
    % Mild wind disturbance
    M_step_scale = 0.0012;    % N.m per normalized paper unit
    M_sine_scale = 0.0008;    % N.m per normalized paper unit
elseif mode == 2
    % Strong paper-like wind disturbance
    M_step_scale = 0.0030;    % N.m per normalized paper unit
    M_sine_scale = 0.0020;    % N.m per normalized paper unit
else
    % Custom/intermediate wind disturbance
    M_step_scale = 0.0020;    % N.m per normalized paper unit
    M_sine_scale = 0.0012;    % N.m per normalized paper unit
end

% ------------------------------------------------------------
% Step/gust pulses at 6, 10, and 15 seconds
% ------------------------------------------------------------
g1 = 0.0;
g2 = 0.0;
g3 = 0.0;

if t >= t1 && t < (t1 + gustWidth)
    g1 = stepAmpPaper;
end

if t >= t2 && t < (t2 + gustWidth)
    g2 = stepAmpPaper;
end

if t >= t3 && t < (t3 + gustWidth)
    g3 = stepAmpPaper;
end

% ------------------------------------------------------------
% 0.5 Hz sinusoidal airflow from 20 s to 30 s
% ------------------------------------------------------------
s = 0.0;
s90 = 0.0;
sSlow = 0.0;

if t >= sineStart && t <= sineEnd
    tau = t - sineStart;
    s = sineAmpPaper * sin(sineOmega*tau);
    s90 = sineAmpPaper * sin(sineOmega*tau + pi/2);
    sSlow = sineAmpPaper * sin(0.70*sineOmega*tau + pi/4);
end

% ------------------------------------------------------------
% Roll, pitch, yaw moment disturbances.
% These three scalar outputs are designed for the existing U2/U3/U4 add blocks.
% ------------------------------------------------------------
d_roll  = factor * (M_step_scale*( g1 - 0.40*g2) + M_sine_scale*s);
d_pitch = factor * (M_step_scale*(-0.50*g1 + g2) + M_sine_scale*s90);
d_yaw   = factor * (M_step_scale*( 0.50*g3) + 0.40*M_sine_scale*sSlow);

% ------------------------------------------------------------
% Keep the existing output names, but now each output is scalar.
% ------------------------------------------------------------
dFxyz        = d_roll;   % existing output port 1 -> U2 disturbance
dMxyz        = d_pitch;  % existing output port 2 -> U3 disturbance
windDisturb6 = d_yaw;    % existing output port 3 -> U4 disturbance

end

== matlab function Adaptive_fuzzy_NTSMC/Planner/MATLAB Function1 ==
  data: t input; slctr input; w input; X0 input; x output; x_d output; x_dd output; y output; y_d output; y_dd output; z output; Tfinal input; z_d output; z_dd output
function [x,x_d,x_dd, y,y_d,y_dd, z,z_d,z_dd] = fcn(t, slctr, w, X0, Tfinal)

% Reference trajectory generator
% x, y, z       = desired position
% x_d, y_d, z_d = desired velocity
% x_dd,y_dd,z_dd = desired acceleration
%
% slctr = 1 : circular trajectory
% slctr = 2 : upward helix
% slctr = 3 : figure-eight trajectory
% else      : fixed point X0

% -----------------------------
% Default trajectory parameters
% -----------------------------
R = 1;              % radius/amplitude, use R = 5 if you want larger path
z_const = 1;        % constant height for circle and figure-eight

wc = 2*pi/5;        % circular trajectory angular speed, paper: 2*pi/5
wh = 2*pi/10;       % helix angular speed
w8 = 2*pi/10;       % figure-eight angular speed

z_start = 0;        % helix starting altitude
z_end = 5;          % helix final altitude

if Tfinal > 0
    vz = (z_end - z_start)/Tfinal;
else
    vz = 0.05;
end

% -----------------------------
% Case 1: Circle
% xd = sin(2*pi*t/5)
% yd = cos(2*pi*t/5)
% zd = 1
% -----------------------------
if slctr == 1

    x = R*sin(wc*t);
    y = R*cos(wc*t);
    z = z_const;

    x_d = R*wc*cos(wc*t);
    y_d = -R*wc*sin(wc*t);
    z_d = 0;

    x_dd = -R*wc^2*sin(wc*t);
    y_dd = -R*wc^2*cos(wc*t);
    z_dd = 0;

% -----------------------------
% Case 2: Upward helix
% x = R*sin(wh*t)
% y = R*cos(wh*t)
% z = z_start + vz*t
% -----------------------------
elseif slctr == 2

    x = R*sin(wh*t);
    y = R*cos(wh*t);
    z = z_start + vz*t;

    x_d = R*wh*cos(wh*t);
    y_d = -R*wh*sin(wh*t);
    z_d = vz;

    x_dd = -R*wh^2*sin(wh*t);
    y_dd = -R*wh^2*cos(wh*t);
    z_dd = 0;

% -----------------------------
% Case 3: Figure-eight trajectory
% x = R*sin(w8*t)
% y = R*sin(2*w8*t)
% z = 1
% -----------------------------
elseif slctr == 3

    x = R*sin(w8*t);
    y = R*sin(2*w8*t);
    z = z_const;

    x_d = R*w8*cos(w8*t);
    y_d = 2*R*w8*cos(2*w8*t);
    z_d = 0;

    x_dd = -R*w8^2*sin(w8*t);
    y_dd = -4*R*w8^2*sin(2*w8*t);
    z_dd = 0;

% -----------------------------
% Fixed point mode
% -----------------------------
else

    x = X0(1);
    y = X0(2);
    z = X0(3);

    x_d = 0;
    y_d = 0;
    z_d = 0;

    x_dd = 0;
    y_dd = 0;
    z_dd = 0;

end

end
